simulink model "UAM_Hexa_PID"  (R2026a)
settings: Solver=ode4  StopTime=1  FixedStep=0.01  MaxStep=1e-3
values from neighbouring files (symbols this model uses):
  ArmConstants = struct('l1_dim', l1_dim,                        'l2_dim', l2_dim,                        'Hexa_to_joint_L', L,                        'Mass1', ml1,                        'Mass2', ml2,                        'Inertia1', Hl1,                        'Inertia2', Hl2,                        'MC1', c1,                        'MC2', c2,                        'Servos', Servos)    [init_model.m]    (also in init_var.m)
  Differentiator = struct('G1', G1 ,     'G2', G2 ,     'Q1', Q1 ,     'Q2', Q2 ,     'w1', w1 ,     'w2', w2 ,     'p1', p1 ,     'p2', p2)    [init_model.m]    (also in init_var.m)
  HexaConstants = struct('Mass', mb,                         'Inertia', J ,                         'allo', allo,                          'invallo', invallo,                         'kT', kT)    [init_model.m]    (also in init_var.m)
settings Model: Creator=Carlos Fabian  LastModifiedBy=Carlos Fabian
settings SolverCC: ZeroCrossAlgorithm=Adaptive
settings DebuggingCC: SignalInfNanChecking=error  IgnoredZcDiagnostic=none
settings ExplorerConfigSet: InternalSimMechanicsExplorerSettings=|
  | <ExplorerConfiguration>
  | 
  |   <canonicalview>default</canonicalview>
  | 
  |   <TilePanel>
  |     <TileInfo>
  |       <Tiles Columns="1" Count="1" Height="465" Rows="1" Width="822">
  |         <Row Weight="1"/>
  |         <Column Weight="1"/>
  |         <Tile Height="1" Width="1" X="0" Y="0"/>
  |       </Tiles>
  |     </TileInfo>
  |     <SceneInfo>
  |       <SceneViewer>
  |         <IsThisViewStd>
  |           <IsStandardView>off</IsStandardView>
  |           <StandardViewName>Front</StandardViewName>
  |         </IsThisViewStd>
  |         <BGColor>
  |           <R>1</R>
  |           <G>1</G>
  |           <B>1</B>
  |           <A>1</A>
  |         </BGColor>
  |         <Camera>
  |           <DoPerspective>off</DoPerspective>
  |           <Position>
  |             <X>-16.441436572758622</X>
  |             <Y>16.2506500104891</Y>
  |             <Z>16.720345739541354</Z>
  |           </Position>
  |           <Center>
  |             <X>-0.069213103553238398</X>
  |             <Y>-0.12157345871628422</Y>
  |             <Z>0.34812227033597537</Z>
  |           </Center>
  |           <Up>
  |             <X>0.40824829046386296</X>
  |             <Y>-0.40824829046386296</Y>
  |             <Z>0.81649658092772615</Z>
  |           </Up>
  |           <XLim>2.7610699582758564</XLim>
  |           <YLim>2.7610699582758564</YLim>
  |           <ViewLimDist>0.01</ViewLimDist>
  |         </Camera>
  |       </SceneViewer>
  |     </SceneInfo>
  |   </TilePanel>
  | 
  |   <MechEditorPanel>
  |     <GfxPanelCameraMap/>
  |     <Cameras/>
  |     <VideoCreator>
  |       <IncludeTiles>All</IncludeTiles>
  |       <IncludeTime>on</IncludeTime>
  |       <IncludeWorldFrame>off</IncludeWorldFrame>
  |       <PlaybackSpeedRatio>1</PlaybackSpeedRatio>
  |       <FrameRate>30</FrameRate>
  |       <FrameSize>auto</FrameSize>
  |       <VideoFormat>UncompressedAVI</VideoFormat>
  |     </VideoCreator>
  |   </MechEditorPanel>
  | 
  |   <PlaybackSettings>
  |     <PlaybackSpeedFactor>8</PlaybackSpeedFactor>
  |   </PlaybackSettings>
  | 
  | </ExplorerConfiguration>

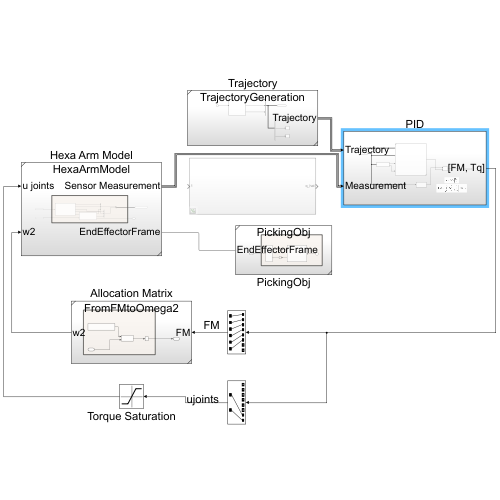
[thumbnail: Simulink's stored preview of the top-level diagram]
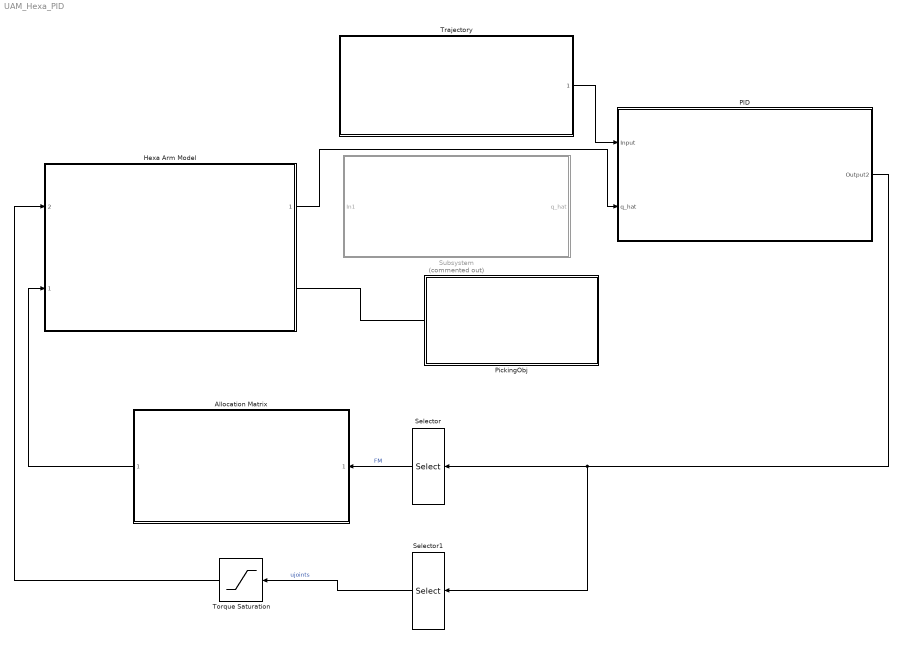
== system UAM_Hexa_PID ==
  Allocation Matrix : Subsystem  ReferencedSubsystem=FromFMtoOmega2
  Hexa Arm Model : Subsystem  ReferencedSubsystem=HexaArmModel
      settings: PortSchema="{\"entries\":[{\"content\":{\"sides\":[{\"content\":{\"connectorIds\":[\"In2\",\"In1\"]},\"type\":\"ConnectorPlacement.EquallySpacedRectSide\",\"uuid\":\"8c321911-c61a-4c60-b031-eeaf4c8b5083\"},{\"content\":{\"connectorIds\":[\"Out1\",\"RConn1\"],\"side\":\"RIGHT\"},\"type\":\"ConnectorPlacement.EquallySpacedRectSide\",\"uuid\":\"3ad1588f-e2f8-4666-8b86-318f5207193d\"},{\"content\":{\"side\":\"TOP\"},\"type\":\"ConnectorPlacement.EquallySpacedRectSide\",\"uuid\":\"710cc49c-59c4-4f69-a558-4588d1d119c0\"}]},\"type\":\"ConnectorPlacement.EquallySpacedConnector\",\"uuid\":\"3e8cca1f-f7f1-4f31-9eba-ef93ff8e81e8\"}],\"packageUris\":[\"http://schema.mathworks.com/mf0/Connector/R2020b\"],\"version\":\"1.0\"}"
  PID : Subsystem
  PickingObj : Subsystem  ReferencedSubsystem=PickingObj
  Selector : Selector  InputPortWidth=8  IndexOptions=Index vector (dialog)  Indices=1:6  OutputSizes=1
  Selector1 : Selector  InputPortWidth=8  IndexOptions=Index vector (dialog)  Indices=7:8  OutputSizes=1
  Subsystem : Subsystem  Commented=on
  Torque Saturation : Saturate  UpperLimit=ArmConstants.Servos.T1max  LowerLimit=-ArmConstants.Servos.T1max
  Trajectory : Subsystem  ReferencedSubsystem=TrajectoryGeneration
  wires:
  Selector/1 -> Allocation Matrix/1  "FM"
  PID/1(Output2) -> Selector/1, Selector1/1
  Torque Saturation/1 -> Hexa Arm Model/2
  Selector1/1 -> Torque Saturation/1  "ujoints"
  Trajectory/1 -> PID/1(Input)
  Allocation Matrix/1 -> Hexa Arm Model/1
  Hexa Arm Model/1 -> PID/2(q_hat)
  connections:
  Hexa Arm Model/RConn1 -- PickingObj/LConn1

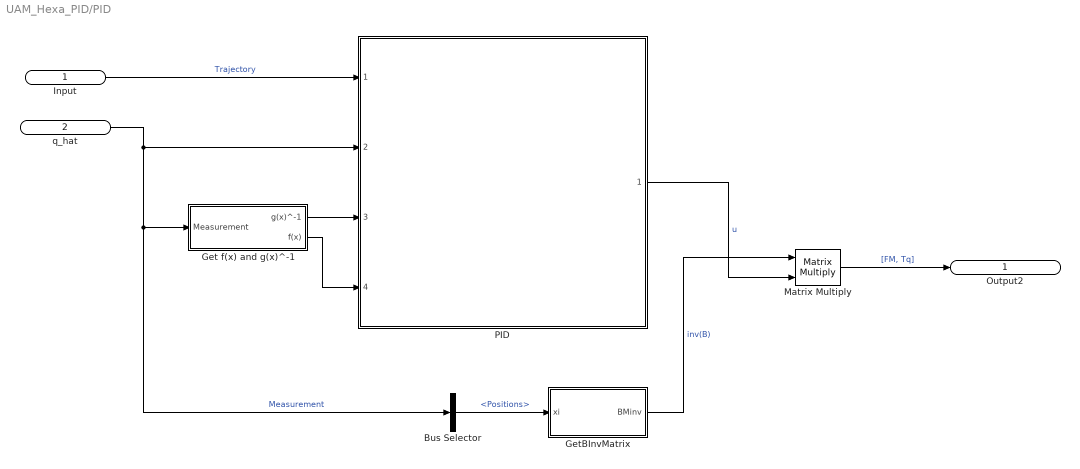
== system UAM_Hexa_PID/PID ==
  Input : Inport
  q_hat : Inport  Port=2
  Bus Selector : BusSelector  OutputSignals=Positions
  Get f(x) and g(x)^-1 : Subsystem
  GetBInvMatrix : MATLAB Function  TreatAsAtomicUnit=on
  Matrix Multiply : Product  Multiplication=Matrix(*)
  PID : Subsystem  ReferencedSubsystem=PIDController
  Output2 : Outport
  wires:
  q_hat/1 -> Get f(x) and g(x)^-1/1(Measurement), Bus Selector/1, PID/2  "Measurement"
  Input/1 -> PID/1  "Trajectory"
  Bus Selector/1 -> GetBInvMatrix/1(xi)  "<Positions>"
  GetBInvMatrix/1(BMinv) -> Matrix Multiply/1  "inv(B)"
  PID/1 -> Matrix Multiply/2  "u"
  Matrix Multiply/1 -> Output2/1  "[FM, Tq]"
  Get f(x) and g(x)^-1/1(g(x)^-1) -> PID/3
  Get f(x) and g(x)^-1/2(f(x)) -> PID/4

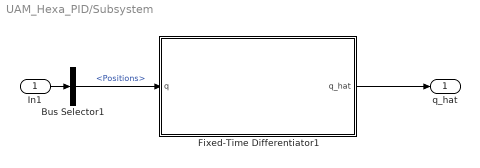
== system UAM_Hexa_PID/Subsystem ==
  In1 : Inport
  Bus Selector1 : BusSelector  OutputSignals=Positions
  Fixed-Time Differentiator1 : Subsystem
      settings: PortSchema="{\"entries\":[{\"content\":{\"sides\":[{\"content\":{\"connectorIds\":[\"Out1\"]},\"type\":\"ConnectorPlacement.EquallySpacedRectSide\",\"uuid\":\"d79ec49c-5563-41e0-ac59-6e897bc19fda\"},{\"content\":{\"connectorIds\":[\"In1\"],\"side\":\"RIGHT\"},\"type\":\"ConnectorPlacement.EquallySpacedRectSide\",\"uuid\":\"1255043e-c90e-4bae-9fb4-4fa06f36f53e\"},{\"content\":{\"side\":\"TOP\"},\"type\":\"ConnectorPlacement.EquallySpacedRectSide\",\"uuid\":\"823ada36-3f22-4ee3-87a1-180276f622bc\"}]},\"type\":\"ConnectorPlacement.EquallySpacedConnector\",\"uuid\":\"7403b609-b333-4977-a854-ed7a71f74338\"}],\"packageUris\":[\"http://schema.mathworks.com/mf0/Connector/R2020b\"],\"version\":\"1.0\"}"
  q_hat : Outport
  wires:
  Bus Selector1/1 -> Fixed-Time Differentiator1/1(q)  "<Positions>"
  Fixed-Time Differentiator1/1(q_hat) -> q_hat/1
  In1/1 -> Bus Selector1/1

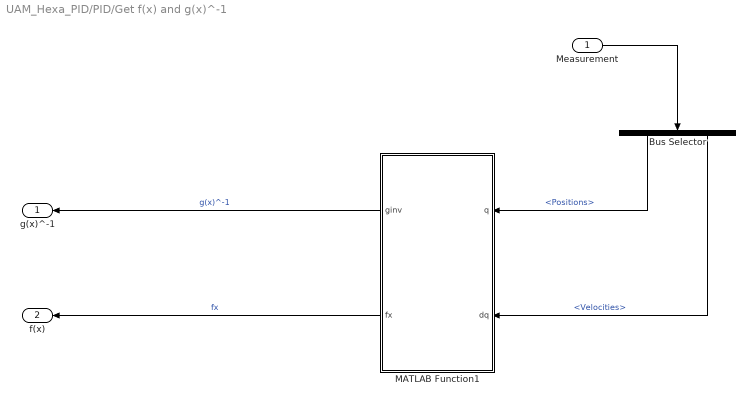
== system UAM_Hexa_PID/PID/Get f(x) and g(x)^-1 ==
  Measurement : Inport
  Bus Selector : BusSelector  OutputSignals=Positions,Velocities
  MATLAB Function1 : MATLAB Function  TreatAsAtomicUnit=on
  g(x)^-1 : Outport
  f(x) : Outport  Port=2
  wires:
  MATLAB Function1/2(fx) -> f(x)/1  "fx"
  MATLAB Function1/1(ginv) -> g(x)^-1/1  "g(x)^-1"
  Measurement/1 -> Bus Selector/1
  Bus Selector/1 -> MATLAB Function1/1(q)  "<Positions>"
  Bus Selector/2 -> MATLAB Function1/2(dq)  "<Velocities>"

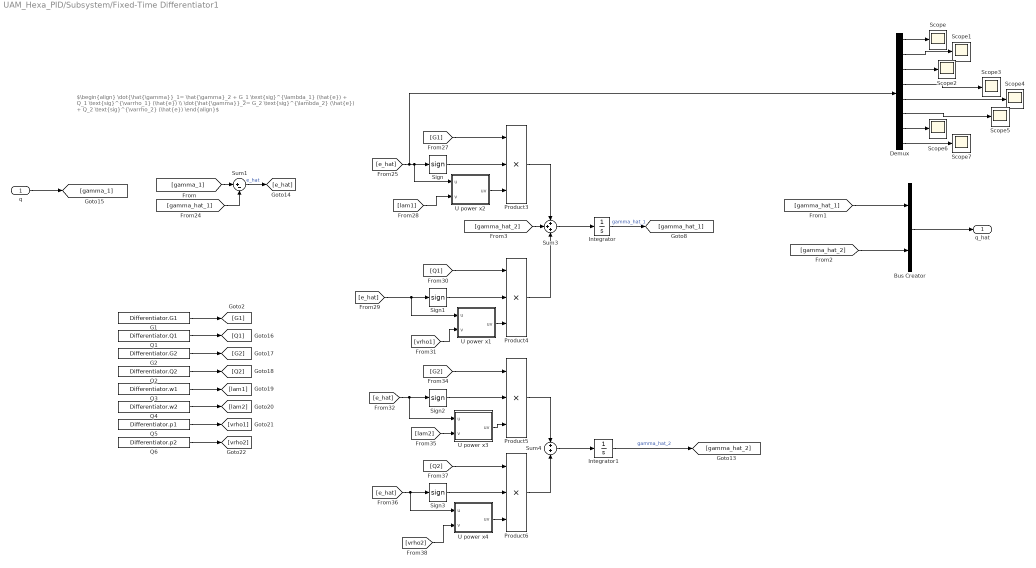
== system UAM_Hexa_PID/Subsystem/Fixed-Time Differentiator1 ==
  note: $\begin{align} \dot{\hat{\gamma}}_1= \hat{\gamma}_2 + G_1 \text{sig}^{\lambda_1} (\hat{e}) + Q_1 \text{sig}^{\varrho_1} (\hat{e}) \\ \dot{\hat{\gamma}}_2= G_2 \text{sig}^{\lambda_2} (\hat{e}) + Q_2 \text{sig}^{\varrho_2} (\hat{e}) \end{align}$
  q : Inport
  Bus Creator : BusCreator  Inputs=2
  Demux : Demux  Outputs=8
  G1 : Constant  Value=Differentiator.G1
  G2 : Constant  Value=Differentiator.G2
  Integrator : Integrator  InitialCondition=[0; 0; 0.23862; 0; 0; 0; 0; 0]  IgnoreLimit=on
  Integrator1 : Integrator  InitialCondition=[0; 0; 0; 0; 0; 0; 0; 0]
  Product{3..6} (4 alike) : Product  Inputs=3
  Q1 : Constant  Value=Differentiator.Q1
  Q2 : Constant  Value=Differentiator.Q2
  Q3 : Constant  Value=Differentiator.w1
  Q4 : Constant  Value=Differentiator.w2
  Q5 : Constant  Value=Differentiator.p1
  Q6 : Constant  Value=Differentiator.p2
  Scope{,1..7} (8 alike) : Scope
      Scope settings: ActiveDisplayYMinimum=0  ActiveDisplayYMaximum=7.1998954942595571E-26
      Scope1 settings: ActiveDisplayYMinimum=-0.00012520279271240959  ActiveDisplayYMaximum=0.00074166117995220127  DataLoggingVariableName=ScopeData4
      Scope2 settings: ActiveDisplayYMinimum=-0.00388840701011419  ActiveDisplayYMaximum=0.034995663091027716  DataLoggingVariableName=ScopeData5
      Scope3 settings: ActiveDisplayYMinimum=-1  ActiveDisplayYMaximum=1  DataLoggingVariableName=ScopeData6
      Scope4 settings: ActiveDisplayYMinimum=-0.0074848921236131578  ActiveDisplayYMaximum=0.00083165468040146177  DataLoggingVariableName=ScopeData7
      Scope5 settings: ActiveDisplayYMinimum=-1  ActiveDisplayYMaximum=1  DataLoggingVariableName=ScopeData8
      Scope6 settings: ActiveDisplayYMinimum=-1  ActiveDisplayYMaximum=1  DataLoggingVariableName=ScopeData9
      Scope7 settings: ActiveDisplayYMinimum=-1  ActiveDisplayYMaximum=1  DataLoggingVariableName=ScopeData10
  Sign{,1..3} (4 alike) : Signum
  Sum1 : Sum  Inputs=|+-
  Sum3 : Sum  Inputs=+++
  Sum4 : Sum  Inputs=+|+
  U power x1 : MATLAB Function  TreatAsAtomicUnit=on
  U power x2 : MATLAB Function  TreatAsAtomicUnit=on
  U power x3 : MATLAB Function  TreatAsAtomicUnit=on
  U power x4 : MATLAB Function  TreatAsAtomicUnit=on
  q_hat : Outport
  wires:
  Product6/1 -> Sum4/2
  G1/1 -> [G1]
  Sum1/1 -> [e_hat]  "e_hat"
  Sign3/1 -> Product6/2
  [gamma_hat_1] -> Sum1/2
  Q5/1 -> [vrho1]
  Q1/1 -> [Q1]
  Q6/1 -> [vrho2]
  [vrho2] -> U power x4/2(v)
  Q2/1 -> [Q2]
  [G1] -> Product3/1
  G2/1 -> [G2]
  Sign2/1 -> Product5/2
  Q4/1 -> [lam2]
  Product5/1 -> Sum4/1
  [gamma_1] -> Sum1/1
  [lam2] -> U power x3/2(v)
  [G2] -> Product5/1
  [Q2] -> Product6/1
  Integrator1/1 -> [gamma_hat_2]  "gamma_hat_2"
  Product3/1 -> Sum3/1
  Sign/1 -> Product3/2
  Q3/1 -> [lam1]
  q/1 -> [gamma_1]
  Integrator/1 -> [gamma_hat_1]  "gamma_hat_1"
  Bus Creator/1 -> q_hat/1
  [gamma_hat_2] -> Bus Creator/2
  Sum4/1 -> Integrator1/1
  Sum3/1 -> Integrator/1
  [gamma_hat_2] -> Sum3/2
  Product4/1 -> Sum3/3
  Sign1/1 -> Product4/2
  [vrho1] -> U power x1/2(v)
  [Q1] -> Product4/1
  [e_hat] -> U power x1/1(u), Sign1/1
  [e_hat] -> U power x3/1(u), Sign2/1
  [e_hat] -> U power x4/1(u), Sign3/1
  [e_hat] -> Demux/1, U power x2/1(u), Sign/1
  U power x2/1(uv) -> Product3/3
  [lam1] -> U power x2/2(v)
  U power x1/1(uv) -> Product4/3
  U power x3/1(uv) -> Product5/3
  U power x4/1(uv) -> Product6/3
  Demux/1 -> Scope/1
  Demux/3 -> Scope2/1
  Demux/2 -> Scope1/1
  Demux/5 -> Scope4/1
  Demux/4 -> Scope3/1
  Demux/6 -> Scope5/1
  Demux/7 -> Scope6/1
  Demux/8 -> Scope7/1
  [gamma_hat_1] -> Bus Creator/1

== matlab function UAM_Hexa_PID/PID/GetBInvMatrix ==
  data: xi input; BMinv output
function BMinv = GetBInvMatrix(xi)

% phi = xi(4);
% th  = xi(5);
% psi = xi(6);
% 
% BM1=[cos(phi)*cos(th),-cos(phi)*sin(psi)+cos(psi)*sin(phi)*sin(th), ...
%     sin(phi)*sin(psi)+cos(phi)*cos(psi)*sin(th),0,0,0;...
%     cos(th)*sin(psi), cos(phi)*cos(psi)+sin(phi)*sin(psi)*sin(th),...
%     -cos(psi)*sin(phi)+cos(phi)*sin(psi)*sin(phi),0,0,0;...
%     -sin(th),cos(th)*sin(psi),cos(phi)*cos(th),0,0,0;...
%     0,0,0,1,sin(phi)*tan(th),cos(phi)*tan(th);...
%     0,0,0,0,cos(phi),-sin(phi);0,0,0,0,sec(th)*sin(phi),cos(phi)*sec(th)];

BM1 = BMatrix(xi);

BM = blkdiag(BM1, eye(2,2));

BMinv = inv(BM);

end

== matlab function UAM_Hexa_PID/Subsystem/Fixed-Time Differentiator1/U power x2 ==
  data: u input; uv output; v input
function uv = u_x(u, v)
i = 1;
uv = zeros(8,1);
if i<9
    absolute = abs(u(i));
    if absolute < 0.0005
        uv(i) = 0;
    else
        uv(i) = absolute ^ v(i);
    end
    i = i + 1;
end
end

== matlab function UAM_Hexa_PID/Subsystem/Fixed-Time Differentiator1/U power x1 ==
  data: u input; uv output; v input
function uv = u_x(u, v)
i = 1;
uv = zeros(8,1);
if i<9
    absolute = abs(u(i));
    if absolute < 0.0005
        uv(i) = 0;
    else
        uv(i) = absolute ^ v(i);
    end
    i = i + 1;
end
end

== matlab function UAM_Hexa_PID/Subsystem/Fixed-Time Differentiator1/U power x3 ==
  data: u input; uv output; v input
function uv = u_x(u, v)
i = 1;
uv = zeros(8,1);
if i<9
    absolute = abs(u(i));
    if absolute < 0.0005
        uv(i) = 0;
    else
        uv(i) = absolute ^ v(i);
    end
    i = i + 1;
end
end

== matlab function UAM_Hexa_PID/Subsystem/Fixed-Time Differentiator1/U power x4 ==
  data: u input; uv output; v input
function uv = u_x(u, v)
i = 1;
uv = zeros(8,1);
if i<9
    absolute = abs(u(i));
    if absolute < 0.0005
        uv(i) = 0;
    else
        uv(i) = absolute ^ v(i);
    end
    i = i + 1;
end
end

== matlab function UAM_Hexa_PID/PID/Get f(x) and g(x)^-1/MATLAB Function1 ==
  data: q input; dq input; HexaConstants parameter; ginv output; fx output; ArmConstants parameter
function [ginv, fx] = Get_DCG_Hexa(q, dq, HexaConstants, ArmConstants)

DM = DMatrix(q, HexaConstants, ArmConstants);
CM = CMatrix(q, dq, HexaConstants, ArmConstants);
Gv = GVector(q, HexaConstants, ArmConstants);

ginv = DM;

fx = DM\( -CM*dq - Gv );

end
